simulink model "QPSK_Carrier_Transmission_Sim"  (R2022a)
settings: Solver=VariableStepAuto  StartTime=0.0  StopTime=100000  RelTol=1e-3
libraries: commdigbbndpm3 x2, commchan3 x1, commsink2 x1, commrandsrc3 x1
settings Model: NumberOfSteps=10000  Creator=Administrator  LastModifiedBy=Administrator
settings ModelReferenceCC: EnableRefExpFcnMdlSchedulingChecks=off
settings RTWCC: Description=Generic Real-Time Target  GPUComputeCapability=5.0

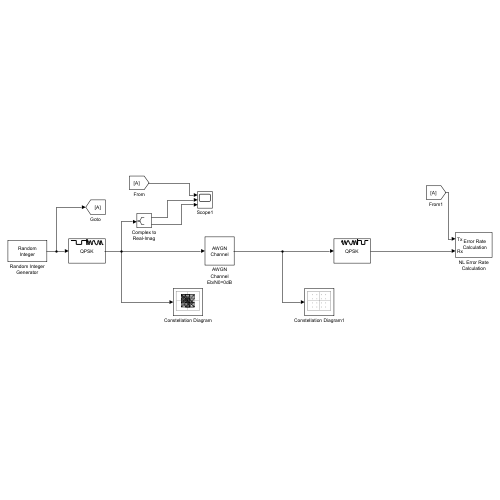
[thumbnail: Simulink's stored preview of the top-level diagram]
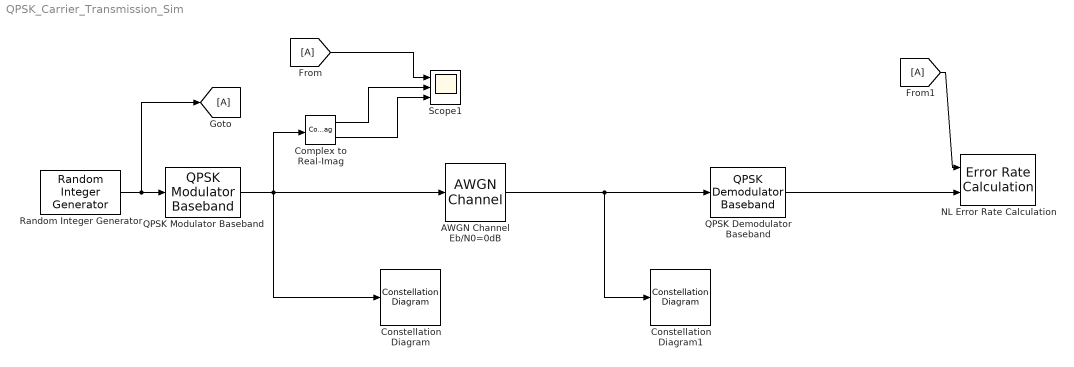
== system QPSK_Carrier_Transmission_Sim ==
  AWGN Channel Eb/N0=0dB : commchan3/AWGN Channel  InputProcessing=Columns as channels (frame based)  noiseMode="Signal to noise ratio  (SNR)"  EbNodB=EsN0  EsNodB=4  SNRdB=10  bitsPerSym=1  Ps=1  Tsym=(1.000000e+00 * 1)  variance=1  seed=67
  Complex to Real-Imag : ComplexToRealImag
  Constellation Diagram : ConstellationDiagram  WindowPosition=[1089.000000,180.000000,917.000000,708.000000,]  Visible=on  ScopeFrameLocation=window  SymbolsToDisplaySource=Property  SymbolsToDisplay=10000  XLimits=[-3.09,3.04]  YLimits=[-1.71,1.53]  ShowTrajectory=on
  Constellation Diagram1 : ConstellationDiagram  WindowPosition=[1.000000,49.000000,1104.000000,924.000000,]  Visible=on  ScopeFrameLocation=window  SymbolsToDisplaySource=Property  SymbolsToDisplay=10000  XLimits=[-1.63,1.63]  YLimits=[-1.38,1.38]
  From : From
  From1 : From
  Goto : Goto
  NL Error Rate Calculation : commsink2/Error Rate Calculation  N=0  st_delay=0  cp_mode=Entire frame  subframe=[]  PMode=Workspace  WsName=ErrorVec  RsMode2=off  stop=off  numErr=100  maxBits=1e6
  QPSK Demodulator Baseband : commdigbbndpm3/QPSK Demodulator Baseband  OutType=Integer  DecType=Hard decision  VarSource=Dialog  Variance=1  Dec=Gray  Ph=pi/4  outDtype1=Inherit via internal rule  outDtype2=Inherit via internal rule  derotateFactorWordLen=16  derotateFactorDataTypeStr=Inherit: Same word length as input  derotateFactorLastDataTypeStr=Inherit: Same word length as input
  QPSK Modulator Baseband : commdigbbndpm3/QPSK Modulator Baseband  InType=Integer  Enc=Gray  Ph=pi/4  outDtype=double  outWordLen=16  outUDDataType=sfix(16)  outFracLenMode=Best precision  outFracLen=15  outDataTypeStr=double  outLastDataTypeStr=double
  Random Integer Generator : commrandsrc3/Random Integer Generator  SetSize=4  SeedSource=Parameter  Seed=37  SampleTime=1  SamplesPerFrame=1  OutputDataType=double  SimulateUsing=Interpreted execution
  Scope1 : Scope  NumInputPorts=3
  wires:
  Random Integer Generator/1 -> Goto/1, QPSK Modulator Baseband/1
  QPSK Modulator Baseband/1 -> Constellation Diagram/1, Complex to Real-Imag/1, AWGN Channel Eb/N0=0dB/1
  AWGN Channel Eb/N0=0dB/1 -> QPSK Demodulator Baseband/1, Constellation Diagram1/1
  QPSK Demodulator Baseband/1 -> NL Error Rate Calculation/2
  Complex to Real-Imag/1 -> Scope1/2
  Complex to Real-Imag/2 -> Scope1/3
  From/1 -> Scope1/1
  From1/1 -> NL Error Rate Calculation/1
